simulink model "launch_chart_check_valid"  (R2022b)
settings: Solver=VariableStepAuto  StartTime=0.0  StopTime=10.0  RelTol=1e-3
settings Model: Creator=22872  LastModifiedBy=22872

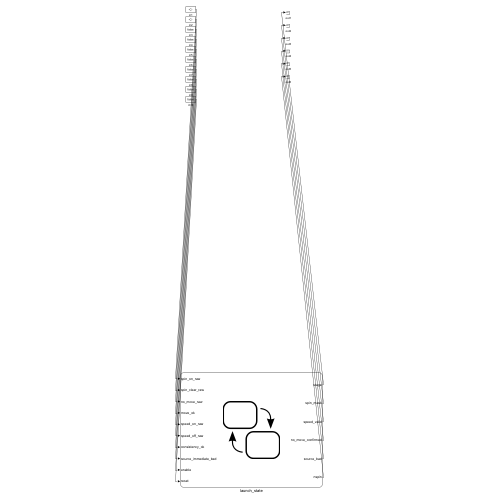
[thumbnail: Simulink's stored preview of the top-level diagram]
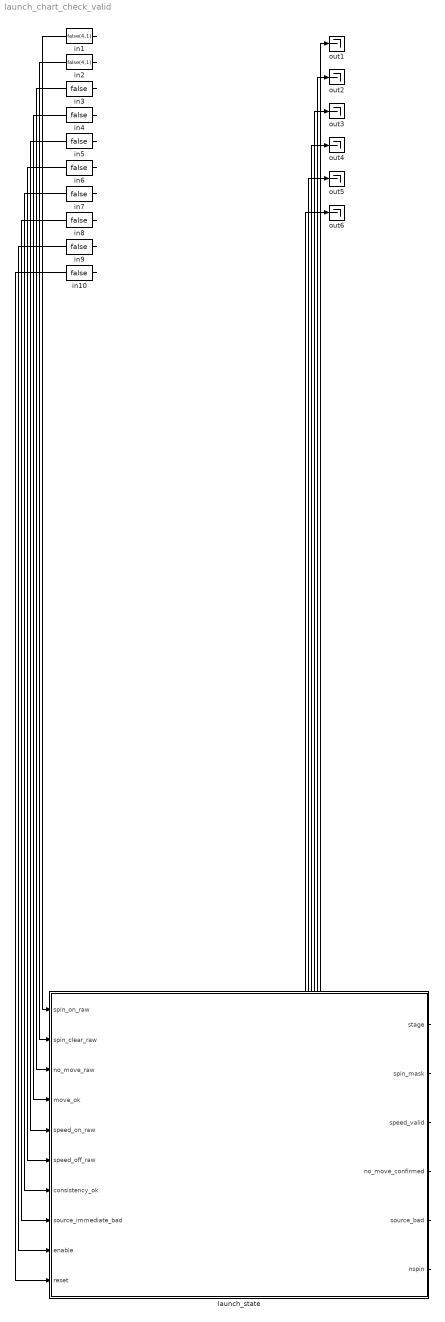
== system launch_chart_check_valid ==
  in1 : Constant  Value=false(4,1)  OutDataTypeStr=boolean
  in{3..10} (8 alike) : Constant  Value=false  OutDataTypeStr=boolean
  in2 : Constant  Value=false(4,1)  OutDataTypeStr=boolean
  launch_state : Stateflow chart  TreatAsAtomicUnit=on
  out{1..6} (6 alike) : Terminator
  wires:
  in1/1 -> launch_state/1(spin_on_raw)
  in2/1 -> launch_state/2(spin_clear_raw)
  in3/1 -> launch_state/3(no_move_raw)
  in4/1 -> launch_state/4(move_ok)
  in5/1 -> launch_state/5(speed_on_raw)
  in6/1 -> launch_state/6(speed_off_raw)
  in7/1 -> launch_state/7(consistency_ok)
  in8/1 -> launch_state/8(source_immediate_bad)
  in9/1 -> launch_state/9(enable)
  in10/1 -> launch_state/10(reset)
  launch_state/1(stage) -> out1/1
  launch_state/2(spin_mask) -> out2/1
  launch_state/3(speed_valid) -> out3/1
  launch_state/4(no_move_confirmed) -> out4/1
  launch_state/5(source_bad) -> out5/1
  launch_state/6(nspin) -> out6/1

== stateflow chart launch_chart_check_valid/launch_state ==
  settings: updateMethod=DISCRETE  sampleTime=0.001
  state MONITOR [parallel]
    entry:
    spin_on_t=zeros(4,1); spin_clear_t=zeros(4,1); spin_mask=false(4,1); nspin=0; no_move_t=0;
    no_move_confirmed=false; speed_on_t=0; speed_off_t=0; speed_valid=false; cons_bad_t=0;
    source_bad=false; desired_stage=uint8(255);
    during:
    if enable<=0.5 || reset>0.5
    spin_on_t=zeros(4,1); spin_clear_t=zeros(4,1); spin_mask=false(4,1); nspin=0; no_move_t=0;
    no_move_confirmed=false; speed_on_t=0; speed_off_t=0; speed_valid=false; cons_bad_t=0;
    source_bad=false; if enable<=0.5, desired_stage=uint8(255); else, desired_stage=uint8(0);
    end
    else
    for i=1:4
    if spin_on_raw(i), spin_on_t(i)=min(P.t_spin_on,spin_on_t(i)+P.Ts); spin_clear_t(i)=0;
    else, spin_on_t(i)=max(0,spin_on_t(i)-P.Ts); if spin_clear_raw(i), spin_clear_t(i)=min(P.t_spin_clear,spin_clear_t(i)+P.Ts);
    else, spin_clear_t(i)=0;
    end, end
    if spin_on_t(i)>=P.t_spin_on, spin_mask(i)=true; end
    if spin_clear_t(i)>=P.t_spin_clear, spin_mask(i)=false; end
    end
    nspin=sum(double(spin_mask));
    if no_move_raw, no_move_t=min(P.t_no_move,no_move_t+P.Ts); elseif move_ok, no_move_t=0; else, no_move_t=max(0,no_move_t-P.Ts); end
    no_move_confirmed=no_move_t>=P.t_no_move;
    if consistency_ok, cons_bad_t=max(0,cons_bad_t-P.Ts); else, cons_bad_t=min(P.t_cons_bad,cons_bad_t+P.Ts); end
    source_bad=source_immediate_bad || cons_bad_t>=P.t_cons_bad;
    if ~speed_valid
    if speed_on_raw && nspin<=1 && ~source_bad, speed_on_t=min(P.t_speed_on,speed_on_t+P.Ts); else, speed_on_t=0; end
    if speed_on_t>=P.t_speed_on, speed_valid=true; speed_off_t=0; end
    else
    if speed_off_raw || nspin>=2 || source_bad, speed_off_t=min(P.t_speed_off,speed_off_t+P.Ts); else, speed_off_t=0; end
    if speed_off_t>=P.t_speed_off, speed_valid=false; speed_on_t=0; end
    end
    if source_bad, desired_stage=uint8(6); elseif nspin>=2, desired_stage=uint8(4);
    elseif nspin==1, desired_stage=uint8(3); elseif speed_valid, desired_stage=uint8(5);
    elseif no_move_confirmed, desired_stage=uint8(2); elseif move_ok, desired_stage=uint8(1);
    else, desired_stage=uint8(0); end
    end
    settings: executionOrder=1
  state MODE [parallel]
    settings: executionOrder=2
    state DISABLED
      entry: stage = uint8(255);
    state START_PROBE
      entry: stage = uint8(0);
    state NORMAL_LAUNCH
      entry: stage = uint8(1);
    state HEAVY_NO_MOVE
      entry: stage = uint8(2);
    state SINGLE_SPIN
      entry: stage = uint8(3);
    state MULTI_SPIN
      entry: stage = uint8(4);
    state WORK_PASS
      entry: stage = uint8(5);
    state PROTECT
      entry: stage = uint8(6);
    (junction 98) -> START_PROBE [order 2] : [desired_stage == uint8(0)]
    (junction 98) -> DISABLED [order 1] : [desired_stage == uint8(255)]
    DISABLED -> (junction 98) : [desired_stage ~= uint8(255)]
    START_PROBE -> (junction 98) : [desired_stage ~= uint8(0)]
    (junction 98) -> HEAVY_NO_MOVE [order 4] : [desired_stage == uint8(2)]
    (junction 98) -> NORMAL_LAUNCH [order 3] : [desired_stage == uint8(1)]
    HEAVY_NO_MOVE -> (junction 98) : [desired_stage ~= uint8(2)]
    NORMAL_LAUNCH -> (junction 98) : [desired_stage ~= uint8(1)]
    (junction 98) -> MULTI_SPIN [order 6] : [desired_stage == uint8(4)]
    (junction 98) -> SINGLE_SPIN [order 5] : [desired_stage == uint8(3)]
    MULTI_SPIN -> (junction 98) : [desired_stage ~= uint8(4)]
    SINGLE_SPIN -> (junction 98) : [desired_stage ~= uint8(3)]
    (junction 98) -> PROTECT [order 8] : [desired_stage == uint8(6)]
    PROTECT -> (junction 98) : [desired_stage ~= uint8(6)]
    (junction 98) -> WORK_PASS [order 7] : [desired_stage == uint8(5)]
    WORK_PASS -> (junction 98) : [desired_stage ~= uint8(5)]
  (default) -> DISABLED
  data: spin_on_raw input boolean size=[4 1]; spin_clear_raw input boolean size=[4 1]; no_move_raw input boolean size=1; move_ok input boolean size=1; speed_on_raw input boolean size=1; speed_off_raw input boolean size=1; consistency_ok input boolean size=1; source_immediate_bad input boolean size=1; enable input boolean size=1; reset input boolean size=1; stage output uint8; spin_mask output boolean size=[4 1]; speed_valid output boolean; no_move_confirmed output boolean; source_bad output boolean; nspin output double; P parameter; spin_on_t local size=[4 1]; spin_clear_t local size=[4 1]; no_move_t local; speed_on_t local; speed_off_t local; cons_bad_t local; desired_stage local uint8; i local double size=1
